simulink model "furuta_hybrid_model"  (R2026b)
settings: Solver=ode23t  StopTime=0.25  MaxStep=5.0000000000000002e-05  RelTol=1e-5  AbsTol=1e-8
model workspace (MAT data in the model file):
  cfg : object (value not decoded)
  disableTime = 100
  drive : object (value not decoded)
  enableTime = 0
  furutaCoverImages : object (value not decoded)
  initialState = [0; 3.14159265359; 0; 0]
  p : object (value not decoded)
symbols that are objects in the model workspace (value not decoded): cfg, drive, p
undefined symbols (not defined in the file): X, Y, Z
libraries: sm_lib x23, nesl_utility x13, fl_lib x8, ee_lib x3
(part 2 of 2)

== matlab function furuta_hybrid_model/Hybrid Controller ==
  data: state input; voltage output; mode input; armReference input; controllerId input; memory input; swing input; energy output; angle output; requestedVoltage output; nextMemory output
function [voltage,energy,angle,requestedVoltage,nextMemory]=controller(state,mode,armReference,controllerId,memory,swing)
p.L0=0.20000000000000001;
p.l1=0.14000000000000001;
p.m1=0.11;
p.J0=0.0070000000000000001;
p.J1cm=0.001;
p.J1ax=1.0000000000000001e-05;
p.b0=0.0011999999999999999;
p.b1=0.00040000000000000002;
p.R=4;
p.Kt=0.035000000000000003;
p.Ke=0.035000000000000003;
p.N=5;
p.eta=0.84999999999999998;
p.g=9.8100000000000005;
cfg.sampleTime=0.0050000000000000001;
cfg.energyGain=100;
cfg.energyOffset=0.040000000000000001;
cfg.armCenterGain=4;
cfg.armDampingGain=3;
cfg.accelerationLimit=25;
cfg.kickAcceleration=3;
cfg.kickRate=0.029999999999999999;
cfg.signSlope=8;
cfg.voltageLimit=12;
cfg.captureAngle=0.31415926535897931;
cfg.captureRate=3;
cfg.captureArmRate=3;
cfg.captureVoltage=10;
cfg.releaseAngle=0.6108652381980153;
cfg.releaseRate=6;
cfg.armLimit=3.1415926535897931;
cfg.speedLimit=20;
controllers.pid.armP=1.6593633925149216;
controllers.pid.pendulumP=38.217129264798913;
controllers.pid.armD=1.4592670795718758;
controllers.pid.pendulumD=4.8323944599812609;
controllers.pid.armI=0.84980172552757549;
controllers.pid.filterRate=80;
controllers.pid.antiWindupRate=5;
controllers.pid.voltageLimit=12;
controllers.pid.initialState=[0;0.087266462599716474;0;0];
controllers.pid.targetPoles=[-1.5 -2 -3 -4 -5];
controllers.lqrK=[-17.188733853924433 -156.4465860723966 -10.60646151205961 -19.680992214292239];
controllers.poleK=[-0.56653448368505022 -32.166364129845277 -0.93582151344960585 -3.9486762492556666];
[voltage,energy,angle,requestedVoltage,nextMemory]=furuta_selected_control(state,mode,armReference,p,cfg,controllers,controllerId,memory,swing);
end
function [voltage,energy,angle,requestedVoltage,nextMemory] = furuta_selected_control(state,mode,armReference,p,cfg,controllers,controllerId,memory,swing)
% Select one stabilization law. Memory contains PID states and previous mode/ID.
if nargin==9 && mode==1
    voltage = swing(1);
    energy = swing(2);
    requestedVoltage = swing(3);
    angle = atan2(sin(state(2)),cos(state(2)));
else
    [voltage,energy,angle,requestedVoltage] = furuta_hybrid_control( ...
        state,mode,armReference,p,cfg,controllers.lqrK);
end
nextMemory = [0;0;0;mode;controllerId];
if mode~=2
    return
end
errorState = [state(1)-armReference;angle;state(3);state(4)];
if controllerId==1
    g = controllers.pid;
    pidState = memory(1:3);
    if memory(4)~=2 || memory(5)~=1
        % Initialize derivatives from the measured rates on entering PID.
        pidState = [0;errorState(1)-state(3)/g.filterRate;angle-state(4)/g.filterRate];
    end
    [voltage,requestedVoltage,derivative] = furuta_pid(errorState(1),angle,pidState,g);
    % Exact low-pass updates and Euler integration of the anti-windup state.
    decay = exp(-g.filterRate*cfg.sampleTime);
    nextMemory(1) = pidState(1)+cfg.sampleTime*derivative(1);
    nextMemory(2:3) = decay*pidState(2:3)+(1-decay)*errorState(1:2);
elseif controllerId==2
    [voltage,requestedVoltage] = furuta_pole_placement(errorState,controllers.poleK,cfg.voltageLimit);
elseif controllerId~=3
    voltage = 0;
    requestedVoltage = 0;
end
end

function [voltage, requestedVoltage, stateDerivative] = furuta_pid(theta0,theta1,state,g)
% Continuous PID/PD controller. State = [integral voltage; filtered angles].
% Initialize state with [0; initial theta0; initial theta1] for each experiment.
armRate = g.filterRate*(theta0-state(2));
pendulumRate = g.filterRate*(theta1-state(3));
requestedVoltage = g.armP*theta0 + state(1) + g.armD*armRate + ...
    g.pendulumP*theta1 + g.pendulumD*pendulumRate;
voltage = min(g.voltageLimit,max(-g.voltageLimit,requestedVoltage));
stateDerivative = [g.armI*theta0 + g.antiWindupRate*(voltage-requestedVoltage); ...
    armRate;pendulumRate];
end

function [voltage,requestedVoltage] = furuta_pole_placement(state,K,voltageLimit)
% State order: theta0, theta1, omega0, omega1 in radians and radians/second.
requestedVoltage = -K*state;
voltage = min(voltageLimit,max(-voltageLimit,requestedVoltage));
end

function [voltage,energy,angle,requestedVoltage] = furuta_hybrid_control(state,mode,armReference,p,cfg,K)
% Mode 1 swings up, mode 2 stabilizes, mode 0 commands zero motor voltage.
angle = atan2(sin(state(2)),cos(state(2)));
Jp = p.J1cm+p.m1*p.l1^2;
energy = 0.5*Jp*state(4)^2+p.m1*p.g*p.l1*cos(state(2));
voltage = 0;
requestedVoltage = 0;
if mode==1
    [voltage,energy,requestedVoltage] = furuta_swingup(state,p,cfg);
elseif mode==2
    errorState = [state(1)-armReference;angle;state(3);state(4)];
    [voltage,requestedVoltage] = furuta_lqr(errorState,K,cfg.voltageLimit);
end
end

function [voltage,energy,requestedVoltage] = furuta_swingup(state,p,cfg)
% Energy shaping produces a desired arm acceleration, mapped to motor voltage.
arm = state(1); pendulum = state(2);
armRate = state(3); pendulumRate = state(4);
c = cos(pendulum);
Jp = p.J1cm+p.m1*p.l1^2;
targetEnergy = p.m1*p.g*p.l1;
energy = 0.5*Jp*pendulumRate^2+targetEnergy*c;
acceleration = cfg.energyGain*(energy-targetEnergy-cfg.energyOffset)* ...
    tanh(cfg.signSlope*pendulumRate*c) ...
    - cfg.armCenterGain*arm-cfg.armDampingGain*armRate;
% Supply an initial push when exactly at rest near the hanging equilibrium.
if abs(pendulumRate)<cfg.kickRate && energy<0
    acceleration = acceleration+cfg.kickAcceleration;
end
acceleration = min(cfg.accelerationLimit,max(-cfg.accelerationLimit,acceleration));
torque = furuta_swingup_torque(state,acceleration,p);
motorGain = p.eta*p.N*p.Kt/p.R;
requestedVoltage = torque/motorGain+p.Ke*p.N*armRate;
voltage = min(cfg.voltageLimit,max(-cfg.voltageLimit,requestedVoltage));
end

function torque = furuta_swingup_torque(state,acceleration,p)
% Invert the provisional swing-up plant for the requested arm acceleration.
s = sin(state(2));
c = cos(state(2));
armRate = state(3);
pendulumRate = state(4);
Jp = p.J1cm+p.m1*p.l1^2;
difference = Jp-p.J1ax;
coupling = p.m1*p.L0*p.l1;
targetEnergy = p.m1*p.g*p.l1;
M11 = p.J0+p.m1*p.L0^2+Jp*s^2+p.J1ax*c^2;
M12 = coupling*c;
velocity0 = 2*difference*s*c*armRate*pendulumRate-coupling*s*pendulumRate^2;
pendulumForce = difference*s*c*armRate^2+targetEnergy*s-p.b1*pendulumRate;
pendulumAcceleration = (pendulumForce-M12*acceleration)/Jp;
torque = M11*acceleration+M12*pendulumAcceleration+velocity0+p.b0*armRate;
end

function [voltage,requestedVoltage] = furuta_lqr(state,K,voltageLimit)
% State order: theta0, theta1, omega0, omega1 in radians and radians/second.
requestedVoltage = -K*state;
voltage = min(voltageLimit,max(-voltageLimit,requestedVoltage));
end

== stateflow chart furuta_hybrid_model/Supervisor ==
  settings: updateMethod=DISCRETE  sampleTime=0.0050000000000000001
  state Swing_Up
    entry:
    mode=1; armReference=0;
    during:
    mode=1;
  state Stabilization
    entry:
    mode=2; armReference=state(1);
    during:
    mode=2;
  state Safe_Stop
    entry:
    mode=0; armReference=0;
    during:
    mode=0;
  Stabilization -> Swing_Up [order 2] : [abs(atan2(sin(state(2)),cos(state(2))))>0.6108652381980153 || abs(state(4))>6]
  (default) -> Swing_Up
  Swing_Up -> Stabilization [order 2] : [abs(atan2(sin(state(2)),cos(state(2))))<0.31415926535897931 && abs(state(4))<3 && abs(state(3))<3 && abs(-156.4465860723966*(atan2(sin(state(2)),cos(state(2))))+-10.60646151205961*state(3)+-19.680992214292239*state(4))<10 && ((controllerId==1 && abs(38.217129264798913*(atan2(sin(state(2)),cos(state(2))))+1.4592670795718758*state(3)+4.8323944599812609*state(4))<10) || (controllerId==2 && abs(-32.166364129845277*(atan2(sin(state(2)),cos(state(2))))+-0.93582151344960585*state(3)+-3.9486762492556666*state(4))<10) || controllerId==3)]
  Swing_Up -> Safe_Stop [order 1] : [enabled<=0 || (controllerId~=1 && controllerId~=2 && controllerId~=3) || any(~isfinite(state)) || abs(state(1))>=3.1415926535897931 || abs(state(3))>=20 || abs(state(4))>=20]
  Stabilization -> Safe_Stop [order 1] : [enabled<=0 || (controllerId~=1 && controllerId~=2 && controllerId~=3) || any(~isfinite(state)) || abs(state(1))>=3.1415926535897931 || abs(state(3))>=20 || abs(state(4))>=20]
  data: state input size=[4 1]; enabled input; controllerId input; mode output; armReference output
